simulink model "Lab1_3_1_2_AccProfile"  (R2024b)
settings: Solver=ode5  StartTime=0.0  StopTime=4  FixedStep=1e-03  RelTol=1e-3
undefined symbols (not defined in the file): Kd, Ki, Kp, Kw, National_Instruments, PCI, rpm2rads, sens, TL
libraries: sldrtlib x2, SignalEditorBlockLib x1
settings Model: SimulationMode=external  ExtModeTrigDuration=45001  Creator=lenovo  LastModifiedBy=aboulenien
settings DataIOCC: ReturnWorkspaceOutputs=off
settings HardwareCC: ProdBitPerLong=64  ProdHWDeviceType=Intel->x86-64 (Linux 64)
settings RTWCC: Description=Simulink Desktop Real-Time  SystemTargetFile=sldrt.tlc  TemplateMakefile=sldrt.tmf  RTWCompilerOptimization=on
settings CodeAppCC: MaxIdLength=95
settings SimulinkDesktopRealTimeCC: TargetLibSuffix=_sldrt.a  TargetPreCompLibLocation=C:\Program Files\MATLAB\R2024b\toolbox\sldrt\lib\win64  ParMdlRefBuildCompliant=on

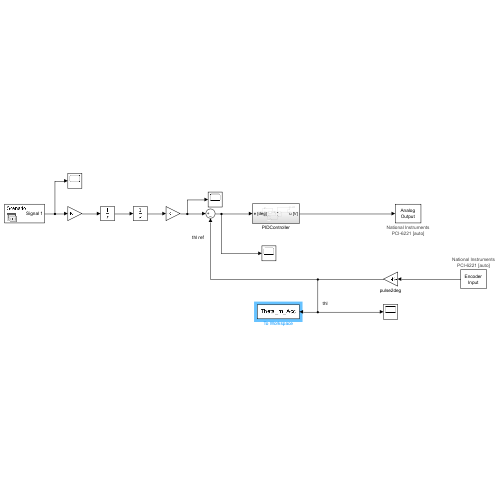
[thumbnail: Simulink's stored preview of the top-level diagram]
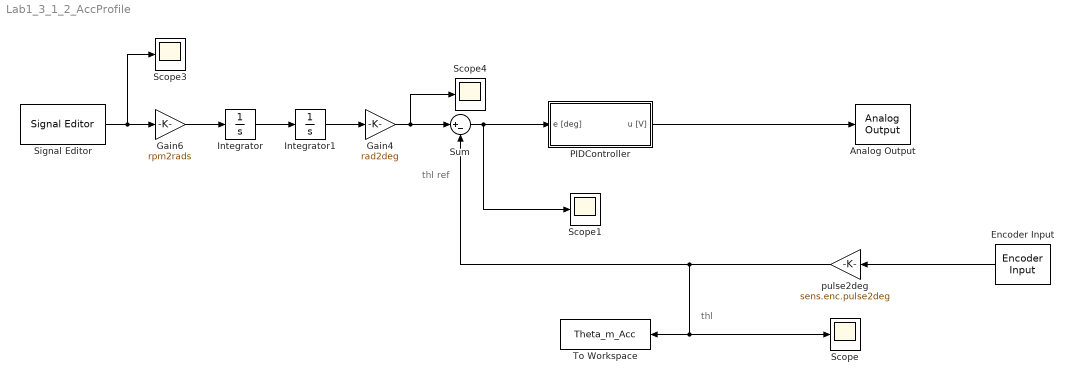
== system Lab1_3_1_2_AccProfile ==
  note: thl
  note: thl ref
  Analog Output : sldrtlib/Analog Output  SampleTime=-1  MaxMissedTicks=10  ShowMissedTicks=off  YieldWhenWaiting=off  DrvName=National_Instruments/PCI-6221  DrvAddress=4294967295  DrvOptions=[0 0 0 2 0]  Channels=1  RangeMode=1  VoltRange=1  InitialValue=0  FinalValue=0
      settings: AttributesFormatString=National Instruments\nPCI-6221 [auto]
  Encoder Input : sldrtlib/Encoder Input  SampleTime=-1  MaxMissedTicks=10  ShowMissedTicks=off  YieldWhenWaiting=off  DrvName=National_Instruments/PCI-6221  DrvAddress=4294967295  DrvOptions=[0 0 0 2 0]  Channels=1  QuadMode=3  IndexPulse=1  InputFilter=Inf  DataType=1
      settings: AttributesFormatString=National Instruments\nPCI-6221 [auto]
  Gain4 : Gain  Gain=rad2deg
  Gain6 : Gain  Gain=rpm2rads
  Integrator : Integrator
  Integrator1 : Integrator
  PIDController : Subsystem
  Scope{,1,3..4} (4 alike) : Scope
  Signal Editor : SignalEditorBlockLib/Signal Editor  FileName=Aprofile.mat  ActiveScenario=Scenario  ActiveSignal=Signal 1  IsBus=off  OutputBusObjectStr=Bus: BusObject  SampleTime=0  Interpolate=off  ZeroCross=off  OutputAfterFinalValue=Setting to zero  Unit=inherit  PreserveSignalName=on  ApplySigPropsToAllScenarios=on  ApplySigPropsToAllSignals=off
  Sum : Sum  Inputs=|+-
  To Workspace : ToWorkspace  VariableName=Theta_m_Acc  SaveFormat=Structure With Time  SampleTime=0.001
  pulse2deg : Gain  Gain=sens.enc.pulse2deg
  wires:
  Integrator1/1 -> Gain4/1
  Integrator/1 -> Integrator1/1
  PIDController/1(u [V]) -> Analog Output/1
  Encoder Input/1 -> pulse2deg/1
  Signal Editor/1 -> Gain6/1, Scope3/1
  Gain6/1 -> Integrator/1
  Gain4/1 -> Scope4/1, Sum/1
  pulse2deg/1 -> To Workspace/1, Scope/1, Sum/2
  Sum/1 -> PIDController/1(e [deg]), Scope1/1

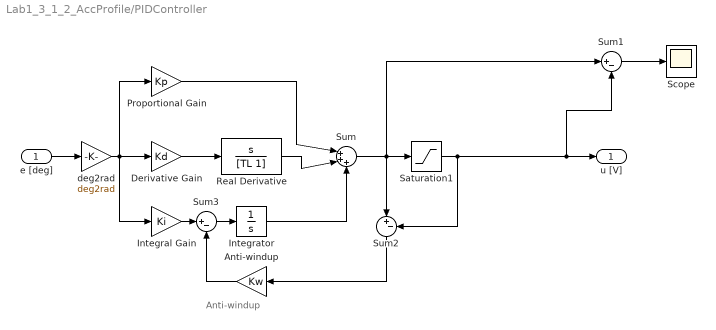
== system Lab1_3_1_2_AccProfile/PIDController ==
  note: Anti-windup
  e [deg] : Inport
  Anti-windup : Gain  Gain=Kw
  Derivative Gain : Gain  Gain=Kd
  Integral Gain : Gain  Gain=Ki
  Integrator : Integrator
  Proportional Gain : Gain  Gain=Kp
  Real Derivative : TransferFcn  Numerator=[1 0]  Denominator=[TL 1]
  Saturation1 : Saturate  UpperLimit=12  LowerLimit=-12
  Scope : Scope
  Sum : Sum  Inputs=|+++
  Sum1 : Sum  Inputs=|+-
  Sum2 : Sum  Inputs=|+-
  Sum3 : Sum  Inputs=|+-
  deg2rad : Gain  Gain=deg2rad
  u [V] : Outport
  wires:
  Saturation1/1 -> Sum2/2, Sum1/2, u [V]/1
  Sum1/1 -> Scope/1
  deg2rad/1 -> Derivative Gain/1, Integral Gain/1, Proportional Gain/1
  e [deg]/1 -> deg2rad/1
  Proportional Gain/1 -> Sum/1
  Derivative Gain/1 -> Real Derivative/1
  Real Derivative/1 -> Sum/2
  Integrator/1 -> Sum/3
  Sum2/1 -> Anti-windup/1
  Integral Gain/1 -> Sum3/1
  Sum3/1 -> Integrator/1
  Anti-windup/1 -> Sum3/2
  Sum/1 -> Sum1/1, Sum2/1, Saturation1/1
